simulink model "sm_car_"  (R2026b)
settings: Solver=ode23t  StopTime=100  MaxStep=0.4  AbsTol=1e-3  EnableMultiTasking=on
PreLoadFcn:
  | % Due to usability issue in Repeating Sequence block
  | warning('off','Simulink:Masking:Invalid');
  | 
  | % Eliminate unnecessary warnings in inactive variants
  | % Warnings generated only if you click through inactive variant
  | warning('off','MATLAB:nonExistentField');
  | warning('off','Simulink:Parameters:BlkParamUndefined');
PostLoadFcn:
  | set_param([bdroot '/Vehicle'],'popup_trailer','Off')
  | warning('off','sm:sli:setup:compile:LocalSolverNotSupported')
  | %sm_car_config_maneuver(bdroot,'WOT Braking');
  | sm_car_config_vehicle(bdroot,'false');
  | sm_car_config_logging(bdroot);
InitFcn:
  | sm_car_config_camera;
  | Vehicle = sm_car_vehcfg_checkConfig(Vehicle);
  | sm_car_check_tire_model(bdroot);
StartFcn:
  | tic;
StopFcn:
  | Elapsed_Sim_Time = toc;
  | % disp(['Elapsed Sim Time = ' num2str(Elapsed_Sim_Time)]);
undefined symbols (not defined in the file or in its folder): acc_theta, accel_ramp_rate, Axle1D, AxleIn, Camera, Control, Driver, Init, Maneuver, Pedal, Scene, ShaftL1, ShaftL2, ShaftR1, ShaftR2, Visual, X, xy_data_car_side, Y, Z
libraries: sm_lib x290, fl_lib x171, nesl_utility x144, simulink x60, simulink_extras x14, sdl_lib x14, SimscapeFluids_lib x7, Damper_Element x4, Tire_1x2x x4, ee_lib x3, Scene_Utilities x3, sharedTrackingLibrary x2
(part 18 of 22)

== system sm_car_/Vehicle/Vehicle/Chassis/Damper/Decoupled/Damper A2 Heave ==
  "Ctrl " : Inport
  Linear : Subsystem  VariantControl=Linear  mask(Linear Damper with Bumpstop){dam_b=Damper.Damping.d.Value, hp_dpr_top=Damper.Damping.sTop.Value, hp_dpr_bot=Damper.Damping.sBottom.Value, bs_lim_upper=Damper.Endstop.xMax.Value, bs_lim_lower=Damper.Endstop.xMin.Value, bs_k_upper=Damper.Endstop.KxMax.Value, bs_k_lower=Damper.Endstop.KxMin.Value, bs_b_upper=Damper.Endstop.dxMax.Value, bs_b_lower=Damper.Endstop.dxMin.Value, bs_region=Damper.Endstop.xTransition.Value}
      mask prompts: dam_b "Damper (N/(m/s))"; hp_dpr_top "HP Damper Top [xyz] (m)"; hp_dpr_bot "HP Damper Bottom [xyz] (m)"; bs_region "Transition Region (m)"
      mask help: Linear damper with bumpstop at top and bottom.
      mask init:
      | dam_x0 = norm(hp_dpr_top - hp_dpr_bot);
      mask TypeOptions dam_b: Damper/D
      mask DialogControl text_bumpstop_upper Prompt: Upper
      mask DialogControl text_bumpstop_lower Prompt: Lower
      mask DialogControl text_bumpstop_limit Prompt: Limit (m)
      mask DialogControl text_bumpstop_k Prompt: Stiffness (N/m)
      mask DialogControl text_bumpstop_b Prompt: Damping  (N/(m/s))
  Nonlinear : Subsystem  VariantControl=Nonlinear  mask(Nonlinear Damper with Bumpstop){velocity_vector=Damper.Damping.vDamper.Value, force_vector=Damper.Damping.fDamper.Value, hp_dpr_top=Damper.Damping.sTop.Value, hp_dpr_bot=Damper.Damping.sBottom.Value, bs_lim_upper=Damper.Endstop.xMax.Value, bs_lim_lower=Damper.Endstop.xMin.Value, bs_k_upper=Damper.Endstop.KxMax.Value, bs_k_lower=Damper.Endstop.KxMin.Value, bs_b_upper=Damper.Endstop.dxMax.Value, bs_b_lower=Damper.Endstop.dxMin.Value, bs_region=Damper.Endstop.xTransition.Value}
      mask prompts: velocity_vector "Velocity vector"; force_vector "Force vector"; hp_dpr_top "HP Damper Top [xyz] (m)"; hp_dpr_bot "HP Damper Bottom [xyz] (m)"; bs_region "Transition Region (m)"
      mask help: Damper with damping coefficient specified as a lookup table in parallel with a bumpstop.
      mask init:
      | dam_x0 = norm(hp_dpr_top - hp_dpr_bot);
      mask TypeOptions velocity_vector: Damper/velocity_vector
      mask TypeOptions force_vector: Damper/force_vector
      mask DialogControl text_bumpstop_upper Prompt: Upper
      mask DialogControl text_bumpstop_lower Prompt: Lower
      mask DialogControl text_bumpstop_limit Prompt: Limit (m)
      mask DialogControl text_bumpstop_k Prompt: Stiffness (N/m)
      mask DialogControl text_bumpstop_b Prompt: Damping  (N/(m/s))
  " R" : PMIOPort  Side=Left
  " C" : PMIOPort  Port=2  Side=Right
  " meas" : Outport  VectorParamsAs1DForOutWhenUnconnected=off

== system sm_car_/Vehicle/Vehicle/Chassis/Damper/Decoupled/Damper A2 Roll ==
  "Ctrl " : Inport
  Linear : Subsystem  VariantControl=Linear  mask(Linear Damper with Bumpstop){dam_b=Damper.Damping.d.Value, hp_dpr_top=Damper.Damping.sTop.Value, hp_dpr_bot=Damper.Damping.sBottom.Value, bs_lim_upper=Damper.Endstop.xMax.Value, bs_lim_lower=Damper.Endstop.xMin.Value, bs_k_upper=Damper.Endstop.KxMax.Value, bs_k_lower=Damper.Endstop.KxMin.Value, bs_b_upper=Damper.Endstop.dxMax.Value, bs_b_lower=Damper.Endstop.dxMin.Value, bs_region=Damper.Endstop.xTransition.Value}
      mask prompts: dam_b "Damper (N/(m/s))"; hp_dpr_top "HP Damper Top [xyz] (m)"; hp_dpr_bot "HP Damper Bottom [xyz] (m)"; bs_region "Transition Region (m)"
      mask help: Linear damper with bumpstop at top and bottom.
      mask init:
      | dam_x0 = norm(hp_dpr_top - hp_dpr_bot);
      mask TypeOptions dam_b: Damper/D
      mask DialogControl text_bumpstop_upper Prompt: Upper
      mask DialogControl text_bumpstop_lower Prompt: Lower
      mask DialogControl text_bumpstop_limit Prompt: Limit (m)
      mask DialogControl text_bumpstop_k Prompt: Stiffness (N/m)
      mask DialogControl text_bumpstop_b Prompt: Damping  (N/(m/s))
  Nonlinear : Subsystem  VariantControl=Nonlinear  mask(Nonlinear Damper with Bumpstop){velocity_vector=Damper.Damping.vDamper.Value, force_vector=Damper.Damping.fDamper.Value, hp_dpr_top=Damper.Damping.sTop.Value, hp_dpr_bot=Damper.Damping.sBottom.Value, bs_lim_upper=Damper.Endstop.xMax.Value, bs_lim_lower=Damper.Endstop.xMin.Value, bs_k_upper=Damper.Endstop.KxMax.Value, bs_k_lower=Damper.Endstop.KxMin.Value, bs_b_upper=Damper.Endstop.dxMax.Value, bs_b_lower=Damper.Endstop.dxMin.Value, bs_region=Damper.Endstop.xTransition.Value}
      mask prompts: velocity_vector "Velocity vector"; force_vector "Force vector"; hp_dpr_top "HP Damper Top [xyz] (m)"; hp_dpr_bot "HP Damper Bottom [xyz] (m)"; bs_region "Transition Region (m)"
      mask help: Damper with damping coefficient specified as a lookup table in parallel with a bumpstop.
      mask init:
      | dam_x0 = norm(hp_dpr_top - hp_dpr_bot);
      mask TypeOptions velocity_vector: Damper/velocity_vector
      mask TypeOptions force_vector: Damper/force_vector
      mask DialogControl text_bumpstop_upper Prompt: Upper
      mask DialogControl text_bumpstop_lower Prompt: Lower
      mask DialogControl text_bumpstop_limit Prompt: Limit (m)
      mask DialogControl text_bumpstop_k Prompt: Stiffness (N/m)
      mask DialogControl text_bumpstop_b Prompt: Damping  (N/(m/s))
  " R" : PMIOPort  Side=Left
  " C" : PMIOPort  Port=2  Side=Right
  " meas" : Outport  VectorParamsAs1DForOutWhenUnconnected=off

== system sm_car_/Vehicle/Vehicle/Chassis/Spring/Decoupled/Spring A1 Heave ==
  "Ctrl " : Inport
  Linear : Subsystem  VariantControl=Linear  mask(Linear Spring){spr_def0=Spring.xPreload.Value, spr_k=Spring.K.Value, spr_hp_top=Spring.sTop.Value, spr_hp_bot=Spring.sBottom.Value}
      mask prompts: spr_def0 "Spring Preload (m)"; spr_k "Spring Rate (N/m)"; spr_hp_top "HP Top [xyz] (m)"; spr_hp_bot "HP Bottom [xyz] (m)"
      mask help: Spring with linear stiffness.
      mask init:
      | spr_len0 = norm(spr_hp_top-spr_hp_bot);
  No Spring : Subsystem  VariantControl=No_Spring  mask(No Spring){}
      mask help: Sensor only
  Nonlinear : Subsystem  VariantControl=Nonlinear  mask(Nonlinear Spring){spr_def0=Spring.xPreload.Value, deformation_vector=Spring.xSpring.Value, force_vector=Spring.fSpring.Value, spr_hp_top=Spring.sTop.Value, spr_hp_bot=Spring.sBottom.Value}
      mask prompts: spr_def0 "Spring Preload (m)"; deformation_vector "Deformation vector"; force_vector "Force vector"; spr_hp_top "HP Top [xyz] (m)"; spr_hp_bot "HP Bottom [xyz] (m)"
      mask help: Spring with stiffness specified by a lookup table.
      mask init:
      | spr_len0 = norm(spr_hp_top-spr_hp_bot);
      mask TypeOptions deformation_vector: Spring/deformation_vector
      mask TypeOptions force_vector: Spring/force_vector
  " R" : PMIOPort  Side=Left
  " C" : PMIOPort  Port=2  Side=Right
  " meas" : Outport  VectorParamsAs1DForOutWhenUnconnected=off

== system sm_car_/Vehicle/Vehicle/Chassis/Spring/Decoupled/Spring A1 Roll ==
  "Ctrl " : Inport
  Linear : Subsystem  VariantControl=Linear  mask(Linear Spring){spr_def0=Spring.xPreload.Value, spr_k=Spring.K.Value, spr_hp_top=Spring.sTop.Value, spr_hp_bot=Spring.sBottom.Value}
      mask prompts: spr_def0 "Spring Preload (m)"; spr_k "Spring Rate (N/m)"; spr_hp_top "HP Top [xyz] (m)"; spr_hp_bot "HP Bottom [xyz] (m)"
      mask help: Spring with linear stiffness.
      mask init:
      | spr_len0 = norm(spr_hp_top-spr_hp_bot);
  No Spring : Subsystem  VariantControl=No_Spring  mask(No Spring){}
      mask help: Sensor only
  Nonlinear : Subsystem  VariantControl=Nonlinear  mask(Nonlinear Spring){spr_def0=Spring.xPreload.Value, deformation_vector=Spring.xSpring.Value, force_vector=Spring.fSpring.Value, spr_hp_top=Spring.sTop.Value, spr_hp_bot=Spring.sBottom.Value}
      mask prompts: spr_def0 "Spring Preload (m)"; deformation_vector "Deformation vector"; force_vector "Force vector"; spr_hp_top "HP Top [xyz] (m)"; spr_hp_bot "HP Bottom [xyz] (m)"
      mask help: Spring with stiffness specified by a lookup table.
      mask init:
      | spr_len0 = norm(spr_hp_top-spr_hp_bot);
      mask TypeOptions deformation_vector: Spring/deformation_vector
      mask TypeOptions force_vector: Spring/force_vector
  " R" : PMIOPort  Side=Left
  " C" : PMIOPort  Port=2  Side=Right
  " meas" : Outport  VectorParamsAs1DForOutWhenUnconnected=off

== system sm_car_/Vehicle/Vehicle/Chassis/Spring/Decoupled/Spring A2 Heave ==
  "Ctrl " : Inport
  Linear : Subsystem  VariantControl=Linear  mask(Linear Spring){spr_def0=Spring.xPreload.Value, spr_k=Spring.K.Value, spr_hp_top=Spring.sTop.Value, spr_hp_bot=Spring.sBottom.Value}
      mask prompts: spr_def0 "Spring Preload (m)"; spr_k "Spring Rate (N/m)"; spr_hp_top "HP Top [xyz] (m)"; spr_hp_bot "HP Bottom [xyz] (m)"
      mask help: Spring with linear stiffness.
      mask init:
      | spr_len0 = norm(spr_hp_top-spr_hp_bot);
  No Spring : Subsystem  VariantControl=No_Spring  mask(No Spring){}
      mask help: Sensor only
  Nonlinear : Subsystem  VariantControl=Nonlinear  mask(Nonlinear Spring){spr_def0=Spring.xPreload.Value, deformation_vector=Spring.xSpring.Value, force_vector=Spring.fSpring.Value, spr_hp_top=Spring.sTop.Value, spr_hp_bot=Spring.sBottom.Value}
      mask prompts: spr_def0 "Spring Preload (m)"; deformation_vector "Deformation vector"; force_vector "Force vector"; spr_hp_top "HP Top [xyz] (m)"; spr_hp_bot "HP Bottom [xyz] (m)"
      mask help: Spring with stiffness specified by a lookup table.
      mask init:
      | spr_len0 = norm(spr_hp_top-spr_hp_bot);
      mask TypeOptions deformation_vector: Spring/deformation_vector
      mask TypeOptions force_vector: Spring/force_vector
  " R" : PMIOPort  Side=Left
  " C" : PMIOPort  Port=2  Side=Right
  " meas" : Outport  VectorParamsAs1DForOutWhenUnconnected=off

== system sm_car_/Vehicle/Vehicle/Chassis/Spring/Decoupled/Spring A2 Roll ==
  "Ctrl " : Inport
  Linear : Subsystem  VariantControl=Linear  mask(Linear Spring){spr_def0=Spring.xPreload.Value, spr_k=Spring.K.Value, spr_hp_top=Spring.sTop.Value, spr_hp_bot=Spring.sBottom.Value}
      mask prompts: spr_def0 "Spring Preload (m)"; spr_k "Spring Rate (N/m)"; spr_hp_top "HP Top [xyz] (m)"; spr_hp_bot "HP Bottom [xyz] (m)"
      mask help: Spring with linear stiffness.
      mask init:
      | spr_len0 = norm(spr_hp_top-spr_hp_bot);
  No Spring : Subsystem  VariantControl=No_Spring  mask(No Spring){}
      mask help: Sensor only
  Nonlinear : Subsystem  VariantControl=Nonlinear  mask(Nonlinear Spring){spr_def0=Spring.xPreload.Value, deformation_vector=Spring.xSpring.Value, force_vector=Spring.fSpring.Value, spr_hp_top=Spring.sTop.Value, spr_hp_bot=Spring.sBottom.Value}
      mask prompts: spr_def0 "Spring Preload (m)"; deformation_vector "Deformation vector"; force_vector "Force vector"; spr_hp_top "HP Top [xyz] (m)"; spr_hp_bot "HP Bottom [xyz] (m)"
      mask help: Spring with stiffness specified by a lookup table.
      mask init:
      | spr_len0 = norm(spr_hp_top-spr_hp_bot);
      mask TypeOptions deformation_vector: Spring/deformation_vector
      mask TypeOptions force_vector: Spring/force_vector
  " R" : PMIOPort  Side=Left
  " C" : PMIOPort  Port=2  Side=Right
  " meas" : Outport  VectorParamsAs1DForOutWhenUnconnected=off

== system sm_car_/Vehicle/Vehicle/Chassis/Spring/Independent/Spring L1 ==
  "Ctrl " : Inport
  Linear : Subsystem  VariantControl=Linear  mask(Linear Spring){spr_def0=Spring.xPreload.Value, spr_k=Spring.K.Value, spr_hp_top=Spring.sTop.Value, spr_hp_bot=Spring.sBottom.Value}
      mask prompts: spr_def0 "Spring Preload (m)"; spr_k "Spring Rate (N/m)"; spr_hp_top "HP Top [xyz] (m)"; spr_hp_bot "HP Bottom [xyz] (m)"
      mask help: Spring with linear stiffness.
      mask init:
      | spr_len0 = norm(spr_hp_top-spr_hp_bot);
  " R" : PMIOPort  Side=Left
  " C" : PMIOPort  Port=2  Side=Right
  " meas" : Outport  VectorParamsAs1DForOutWhenUnconnected=off

== system sm_car_/Vehicle/Vehicle/Chassis/Spring/Independent/Spring L2 ==
  "Ctrl " : Inport
  Linear : Subsystem  VariantControl=Linear  mask(Linear Spring){spr_def0=Spring.xPreload.Value, spr_k=Spring.K.Value, spr_hp_top=Spring.sTop.Value, spr_hp_bot=Spring.sBottom.Value}
      mask prompts: spr_def0 "Spring Preload (m)"; spr_k "Spring Rate (N/m)"; spr_hp_top "HP Top [xyz] (m)"; spr_hp_bot "HP Bottom [xyz] (m)"
      mask help: Spring with linear stiffness.
      mask init:
      | spr_len0 = norm(spr_hp_top-spr_hp_bot);
  " R" : PMIOPort  Side=Left
  " C" : PMIOPort  Port=2  Side=Right
  " meas" : Outport  VectorParamsAs1DForOutWhenUnconnected=off

== system sm_car_/Vehicle/Vehicle/Chassis/Spring/Independent/Spring R1 ==
  "Ctrl " : Inport
  Linear : Subsystem  VariantControl=Linear  mask(Linear Spring){spr_def0=Spring.xPreload.Value, spr_k=Spring.K.Value, spr_hp_top=Spring.sTop.Value, spr_hp_bot=Spring.sBottom.Value}
      mask prompts: spr_def0 "Spring Preload (m)"; spr_k "Spring Rate (N/m)"; spr_hp_top "HP Top [xyz] (m)"; spr_hp_bot "HP Bottom [xyz] (m)"
      mask help: Spring with linear stiffness.
      mask init:
      | spr_len0 = norm(spr_hp_top-spr_hp_bot);
  " R" : PMIOPort  Side=Left
  " C" : PMIOPort  Port=2  Side=Right
  " meas" : Outport  VectorParamsAs1DForOutWhenUnconnected=off

== system sm_car_/Vehicle/Vehicle/Chassis/Spring/Independent/Spring R2 ==
  "Ctrl " : Inport
  Linear : Subsystem  VariantControl=Linear  mask(Linear Spring){spr_def0=Spring.xPreload.Value, spr_k=Spring.K.Value, spr_hp_top=Spring.sTop.Value, spr_hp_bot=Spring.sBottom.Value}
      mask prompts: spr_def0 "Spring Preload (m)"; spr_k "Spring Rate (N/m)"; spr_hp_top "HP Top [xyz] (m)"; spr_hp_bot "HP Bottom [xyz] (m)"
      mask help: Spring with linear stiffness.
      mask init:
      | spr_len0 = norm(spr_hp_top-spr_hp_bot);
  " R" : PMIOPort  Side=Left
  " C" : PMIOPort  Port=2  Side=Right
  " meas" : Outport  VectorParamsAs1DForOutWhenUnconnected=off

== system sm_car_/Vehicle/Vehicle/Powertrain/Driveline/L2 R2/Sensing Torque L1 ==
  Ideal Torque Sensor : fl_lib/Mechanical/Mechanical Sensors/Ideal Torque Sensor
  PS-Simulink Converter : nesl_utility/PS-Simulink Converter  PhysicalDomain=network_engine_domain  SubClassName=ps_output  LeftPortType=input  RightPortType=output  PseudoPeriodic=off  Frequencies=[]  VectorFormat=1-D array  Unit=N*m  AffineConversion=off
  C : PMIOPort  Side=Right
  R : PMIOPort  Port=2  Side=Left
  M : Outport  VectorParamsAs1DForOutWhenUnconnected=off
  wires:
  PS-Simulink Converter/1 -> M/1
  connections:
  Ideal Torque Sensor/RConn1 -- C/RConn1
  R/RConn1 -- Ideal Torque Sensor/LConn1
  Ideal Torque Sensor/RConn2 -- PS-Simulink Converter/LConn1

== system sm_car_/Vehicle/Vehicle/Powertrain/Driveline/L2 R2/Sensing Torque L2 ==
  Ideal Torque Sensor : fl_lib/Mechanical/Mechanical Sensors/Ideal Torque Sensor
  PS-Simulink Converter : nesl_utility/PS-Simulink Converter  PhysicalDomain=network_engine_domain  SubClassName=ps_output  LeftPortType=input  RightPortType=output  PseudoPeriodic=off  Frequencies=[]  VectorFormat=1-D array  Unit=N*m  AffineConversion=off
  C : PMIOPort  Side=Right
  R : PMIOPort  Port=2  Side=Left
  M : Outport  VectorParamsAs1DForOutWhenUnconnected=off
  wires:
  PS-Simulink Converter/1 -> M/1
  connections:
  Ideal Torque Sensor/RConn2 -- PS-Simulink Converter/LConn1
  R/RConn1 -- Ideal Torque Sensor/LConn1
  Ideal Torque Sensor/RConn1 -- C/RConn1

== system sm_car_/Vehicle/Vehicle/Powertrain/Driveline/L2 R2/Sensing Torque R1 ==
  Ideal Torque Sensor : fl_lib/Mechanical/Mechanical Sensors/Ideal Torque Sensor
  PS-Simulink Converter : nesl_utility/PS-Simulink Converter  PhysicalDomain=network_engine_domain  SubClassName=ps_output  LeftPortType=input  RightPortType=output  PseudoPeriodic=off  Frequencies=[]  VectorFormat=1-D array  Unit=N*m  AffineConversion=off
  C : PMIOPort  Side=Right
  R : PMIOPort  Port=2  Side=Left
  M : Outport  VectorParamsAs1DForOutWhenUnconnected=off
  wires:
  PS-Simulink Converter/1 -> M/1
  connections:
  Ideal Torque Sensor/RConn2 -- PS-Simulink Converter/LConn1
  R/RConn1 -- Ideal Torque Sensor/LConn1
  Ideal Torque Sensor/RConn1 -- C/RConn1

== system sm_car_/Vehicle/Vehicle/Powertrain/Driveline/L2 R2/Sensing Torque R2 ==
  Ideal Torque Sensor : fl_lib/Mechanical/Mechanical Sensors/Ideal Torque Sensor
  PS-Simulink Converter : nesl_utility/PS-Simulink Converter  PhysicalDomain=network_engine_domain  SubClassName=ps_output  LeftPortType=input  RightPortType=output  PseudoPeriodic=off  Frequencies=[]  VectorFormat=1-D array  Unit=N*m  AffineConversion=off
  C : PMIOPort  Side=Right
  R : PMIOPort  Port=2  Side=Left
  M : Outport  VectorParamsAs1DForOutWhenUnconnected=off
  wires:
  PS-Simulink Converter/1 -> M/1
  connections:
  Ideal Torque Sensor/RConn1 -- C/RConn1
  R/RConn1 -- Ideal Torque Sensor/LConn1
  Ideal Torque Sensor/RConn2 -- PS-Simulink Converter/LConn1

== system sm_car_/Vehicle/Vehicle/Powertrain/Driveline/L2 R2/ShaftL1 ==
  Driveshaft Measurements : Subsystem
  Ideal Torque Sensor : fl_lib/Mechanical/Mechanical Sensors/Ideal Torque Sensor
  No Open Connection : sm_lib/Frames and Transforms/Reference Frame
  PS Terminator : fl_lib/Physical Signals/Sinks/PS Terminator
  Simscape Bus B : SimscapeBus  HierarchyStrings=AxleIn;Axle1D
  Simscape Bus Shaft : SimscapeBus  HierarchyStrings=Shaft1D
  Diff : PMIOPort  Side=Right
  B : PMIOPort  Port=2  Side=Left
  meas : Outport  VectorParamsAs1DForOutWhenUnconnected=off
  wires:
  Driveshaft Measurements/1(meas) -> meas/1
  connections:
  Simscape Bus B/LConn2 -- Ideal Torque Sensor/LConn1
  Ideal Torque Sensor/RConn1 -- Simscape Bus Shaft/LConn1
  Diff/RConn1 -- Simscape Bus Shaft/RConn1
  Ideal Torque Sensor/RConn2 -- PS Terminator/LConn1
  B/RConn1 -- Simscape Bus B/RConn1
  No Open Connection/RConn1 -- Simscape Bus B/LConn1

== system sm_car_/Vehicle/Vehicle/Powertrain/Driveline/L2 R2/ShaftL2 ==
  Ideal Rotational Motion Sensor : fl_lib/Mechanical/Mechanical Sensors/Ideal Rotational Motion Sensor  reference=foundation.enum.MeasurementReference.difference  acceleration_port=false  velocity_port=true  position_port=false  wrap_angle=false  offset=0 rad
  Ideal Torque Sensor : fl_lib/Mechanical/Mechanical Sensors/Ideal Torque Sensor
  Mechanical Rotational Reference : fl_lib/Mechanical/Rotational Elements/Mechanical Rotational Reference
  No Open Connection : sm_lib/Frames and Transforms/Reference Frame
  PS-Simulink Converter : nesl_utility/PS-Simulink Converter  PhysicalDomain=network_engine_domain  SubClassName=ps_output  LeftPortType=input  RightPortType=output  PseudoPeriodic=off  Frequencies=[]  VectorFormat=inherit  Unit=inherit  AffineConversion=off
  PS-Simulink Converter1 : nesl_utility/PS-Simulink Converter  PhysicalDomain=network_engine_domain  SubClassName=ps_output  LeftPortType=input  RightPortType=output  PseudoPeriodic=off  Frequencies=[]  VectorFormat=inherit  Unit=inherit  AffineConversion=off
  Simscape Bus B : SimscapeBus  HierarchyStrings=AxleIn;Axle1D
  Simscape Bus Shaft : SimscapeBus  HierarchyStrings=Shaft1D
  Diff : PMIOPort  Side=Right
  B : PMIOPort  Port=2  Side=Left
  Out Bus Element : Outport  PortName=meas  Element=T
  Out Bus Element1 : Outport  PortName=meas  Element=w
  wires:
  PS-Simulink Converter/1 -> Out Bus Element1/1
  PS-Simulink Converter1/1 -> Out Bus Element/1
  connections:
  Simscape Bus B/LConn2 -- Ideal Rotational Motion Sensor/LConn1 -- Ideal Torque Sensor/LConn1
  Ideal Torque Sensor/RConn1 -- Simscape Bus Shaft/LConn1
  Diff/RConn1 -- Simscape Bus Shaft/RConn1
  Ideal Torque Sensor/RConn2 -- PS-Simulink Converter1/LConn1
  B/RConn1 -- Simscape Bus B/RConn1
  No Open Connection/RConn1 -- Simscape Bus B/LConn1
  Ideal Rotational Motion Sensor/RConn1 -- Mechanical Rotational Reference/LConn1
  Ideal Rotational Motion Sensor/RConn2 -- PS-Simulink Converter/LConn1

== system sm_car_/Vehicle/Vehicle/Powertrain/Driveline/L2 R2/ShaftR1 ==
  Driveshaft Measurements : Subsystem
  Ideal Torque Sensor : fl_lib/Mechanical/Mechanical Sensors/Ideal Torque Sensor
  No Open Connection : sm_lib/Frames and Transforms/Reference Frame
  PS Terminator : fl_lib/Physical Signals/Sinks/PS Terminator
  Simscape Bus B : SimscapeBus  HierarchyStrings=AxleIn;Axle1D
  Simscape Bus Shaft : SimscapeBus  HierarchyStrings=Shaft1D
  Diff : PMIOPort  Side=Right
  B : PMIOPort  Port=2  Side=Left
  meas : Outport  VectorParamsAs1DForOutWhenUnconnected=off
  wires:
  Driveshaft Measurements/1(meas) -> meas/1
  connections:
  Simscape Bus B/LConn2 -- Ideal Torque Sensor/LConn1
  Ideal Torque Sensor/RConn1 -- Simscape Bus Shaft/LConn1
  Diff/RConn1 -- Simscape Bus Shaft/RConn1
  Ideal Torque Sensor/RConn2 -- PS Terminator/LConn1
  B/RConn1 -- Simscape Bus B/RConn1
  No Open Connection/RConn1 -- Simscape Bus B/LConn1

== system sm_car_/Vehicle/Vehicle/Powertrain/Driveline/L2 R2/ShaftR2 ==
  Ideal Rotational Motion Sensor : fl_lib/Mechanical/Mechanical Sensors/Ideal Rotational Motion Sensor  reference=foundation.enum.MeasurementReference.difference  acceleration_port=false  velocity_port=true  position_port=false  wrap_angle=false  offset=0 rad
  Ideal Torque Sensor : fl_lib/Mechanical/Mechanical Sensors/Ideal Torque Sensor
  Mechanical Rotational Reference : fl_lib/Mechanical/Rotational Elements/Mechanical Rotational Reference
  No Open Connection : sm_lib/Frames and Transforms/Reference Frame
  PS-Simulink Converter : nesl_utility/PS-Simulink Converter  PhysicalDomain=network_engine_domain  SubClassName=ps_output  LeftPortType=input  RightPortType=output  PseudoPeriodic=off  Frequencies=[]  VectorFormat=inherit  Unit=inherit  AffineConversion=off
  PS-Simulink Converter1 : nesl_utility/PS-Simulink Converter  PhysicalDomain=network_engine_domain  SubClassName=ps_output  LeftPortType=input  RightPortType=output  PseudoPeriodic=off  Frequencies=[]  VectorFormat=inherit  Unit=inherit  AffineConversion=off
  Simscape Bus B : SimscapeBus  HierarchyStrings=AxleIn;Axle1D
  Simscape Bus Shaft : SimscapeBus  HierarchyStrings=Shaft1D
  Diff : PMIOPort  Side=Right
  B : PMIOPort  Port=2  Side=Left
  Out Bus Element : Outport  PortName=meas  Element=T
  Out Bus Element1 : Outport  PortName=meas  Element=w
  wires:
  PS-Simulink Converter/1 -> Out Bus Element1/1
  PS-Simulink Converter1/1 -> Out Bus Element/1
  connections:
  Simscape Bus B/LConn2 -- Ideal Rotational Motion Sensor/LConn1 -- Ideal Torque Sensor/LConn1
  Ideal Torque Sensor/RConn1 -- Simscape Bus Shaft/LConn1
  Diff/RConn1 -- Simscape Bus Shaft/RConn1
  Ideal Torque Sensor/RConn2 -- PS-Simulink Converter1/LConn1
  B/RConn1 -- Simscape Bus B/RConn1
  No Open Connection/RConn1 -- Simscape Bus B/LConn1
  Ideal Rotational Motion Sensor/RConn2 -- PS-Simulink Converter/LConn1
  Ideal Rotational Motion Sensor/RConn1 -- Mechanical Rotational Reference/LConn1

== system sm_car_/Vehicle/Vehicle/Powertrain/Power/Electric L2 R2/Battery ==
  Battery : batteryecm_lib/Battery (Table-Based)  SOC_vec=Power.Battery.vNoLoad.SOC.Value  T_dependence=simscape.enum.tablebattery.temperature_dependence.yes  prm_dir=simscape.enum.tablebattery.prm_dir.noCurrentDirectionality  T_vec=Power.Battery.vNoLoad.T.Value K  V0_mat=Power.Battery.vNoLoad.V0.Value V  V0_vec=[3.1, 3.27, 3.31, 3.5] V  V_range=[0, inf] V  R0_mat=Power.Battery.rTerminal.R0.Value Ohm  R0_vec=[.015, .017, .012, .013] Ohm  R0_dis_mat=[.03, .015, .002; .04, .017, .008; .039, .012, .006; .027, .013, .021] Ohm  R0_dis_vec=[.015, .017, .012, .013] Ohm  R0_ch_mat=[.03, .015, .002; .04, .017, .008; .039, .012, .006; .027, .013, .021] Ohm  R0_ch_vec=[.015, .017, .012, .013] Ohm  AH=Power.Battery.AhTable.Ah.Value hr*A  prm_leak=1  Rleak_vec=[8000, 7000, 6000] Ohm  Rleak=7e3 Ohm  extrapolation_option=simscape.enum.extrapolation.linear  SOC_port=simscape.enum.tablebattery.enable.yes  prm_dyn=simscape.enum.tablebattery.prm_dyn.off  R1_mat=[.089, .076, .01; .042, .022, .099; .019, .007, .002; .051, .043, .029] Ohm  R1_vec=[.076, .022, .007, .043] Ohm  tau1_mat=[44, 148, 235; 93, 110, 1000; 19, 27, 133; .5, 22, 3] s  tau1_vec=[148, 110, 27, 22] s  R2_mat=[.014, .382, .407; .028, .006, .007; .014, .007, .006; .333, .956, .912] Ohm  R2_vec=[.382, .006, .007, .956] Ohm  tau2_mat=[1, 44, 5644; 11, 24, 506; 2, 14, 330; 3310, 13419, 30216] s  tau2_vec=[44, 24, 14, 13419] s  R3_mat=[.014, .382, .407; .028, .006, .007; .014, .007, .006; .333, .956, .912] Ohm  R3_vec=[.382, .006, .007, .956] Ohm  tau3_mat=[1, 44, 5644; 11, 24, 506; 2, 14, 330; 3310, 13419, 30216] s  tau3_vec=[44, 24, 14, 13419] s  R4_mat=[.014, .382, .407; .028, .006, .007; .014, .007, .006; .333, .956, .912] Ohm  R4_vec=[.382, .006, .007, .956] Ohm  tau4_mat=[1, 44, 5644; 11, 24, 506; 2, 14, 330; 3310, 13419, 30216] s  tau4_vec=[44, 24, 14, 13419] s  R5_mat=[.014, .382, .407; .028, .006, .007; .014, .007, .006; .333, .956, .912] Ohm  R5_vec=[.382, .006, .007, .956] Ohm  tau5_mat=[1, 44, 5644; 11, 24, 506; 2, 14, 330; 3310, 13419, 30216] s  tau5_vec=[44, 24, 14, 13419] s  prm_fade=simscape.enum.tablebattery.prm_fade.equations  N0=100  dV0=0  dR0=0  dAH=0  dRleak=0  dR1=0  dR2=0  dR3=0  dR4=0  dR5=0  N0vec=[100, 200, 300]  Tfadevec=[298.15, 323.15] K  dV0vec=[0, 0, 0]  dR0vec=[0, 0, 0]  dAHvec=[0, 0, 0]  dRleakvec=[0, 0, 0]  dR1vec=[0, 0, 0]  dR2vec=[0, 0, 0]  dR3vec=[0, 0, 0]  dR4vec=[0, 0, 0]  dR5vec=[0, 0, 0]  dV0mat=[0, 0; 0, 0; 0, 0]  dR0mat=[0, 0; 0, 0; 0, 0]  dAHmat=[0, 0; 0, 0; 0, 0]  dRleakmat=[0, 0; 0, 0; 0, 0]  dR1mat=[0, 0; 0, 0; 0, 0]  dR2mat=[0, 0; 0, 0; 0, 0]  dR3mat=[0, 0; 0, 0; 0, 0]  dR4mat=[0, 0; 0, 0; 0, 0]  dR5mat=[0, 0; 0, 0; 0, 0]  prm_age_modeling=simscape.enum.tablebattery.prm_age_modeling.equation  storage_dt_age_vec=[0] d  storage_T_age_vec=[273] K  prm_age_OCV=simscape.enum.tablebattery.prm_age_OCV.OCV  OCV_age=0.9  SOC_age=0.6  prm_age_resistance=simscape.enum.tablebattery.prm_age.disabled  OCV_scaling_age_resistance=2.2134e6  OCV_offset_age_resistance=1.632e6  temp_exp_age_resistance=0.515833569 V  t_exp_age_resistance=0.75  T_age_vec_resistance=[273.15, 298.15, 323.15] K  dt_age_vec_resistance=[90, 180, 270, 360] d  dR0_age_vec=[0, 0, 0]  t_meas_dR0_age=100 d  dR0_age_mat=[0, 0, 0; 0, 0, 0; 0, 0, 0; 0, 0, 0]  prm_age_capacity=simscape.enum.tablebattery.prm_age.disabled  OCV_scaling_age_capacity=1.5097e07  OCV_offset_age_capacity=8.3625e06  temp_exp_age_capacity=0.6011 V  t_exp_age_capacity=0.75  T_age_vec_capacity=[273.15, 298.15, 323.15] K  dt_age_vec_capacity=[90, 180, 270, 360] d  dAH_age_vec=[0, 0, 0]  t_meas_dAH_age=100 d  dAH_age_mat=[0, 0, 0; 0, 0, 0; 0, 0, 0; 0, 0, 0]  thermal_port=simscape.enum.thermaleffects.model  temperature=300 K  thermal_mass=30000 J/K  i_specify=off  i_priority=None  i=0 A  i_nominal_specify=off  i_nominal_value=1  i_nominal_unit=A  v_specify=off  v_priority=None  v=0 V  v_nominal_specify=off  v_nominal_value=1  v_nominal_unit=V  stateOfCharge_specify=on  stateOfCharge_priority=High  stateOfCharge=Power.Battery.SOCInit.Value  stateOfCharge_nominal_specify=off  stateOfCharge_nominal_value=1  stateOfCharge_nominal_unit=1  num_cycles_specify=off  num_cycles_priority=High  num_cycles=0  num_cycles_nominal_specify=off  num_cycles_nominal_value=1  num_cycles_nominal_unit=1  cell_temperature_specify=on  cell_temperature_priority=High  cell_temperature=300 K  cell_temperature_nominal_specify=off  cell_temperature_nominal_value=1  cell_temperature_nominal_unit=K
  Bus Selector : BusSelector  OutputSignals=i,v
  DC-DC Converter : ee_lib/Semiconductors & Converters/Converters/DC-DC Converter  Vref_option=ee.enum.converters.voltageref.internal  v_ref=Power.Converter.vRef.Value V  P_rated=Power.Converter.Power.Value W  droop_enabled=true  droop_param=1  droop=0.001*0 V/A  droop_percent=2  Vref_droop=10 V  reversible=1  G_diode=1e-8 1/Ohm  P_fixed=1 W  losses_option=ee.enum.converters.lossesOption.proportionalToSquaredCurrent  eff_rated=Power.Converter.efficiency.Value  tableOption=ee.enum.converters.lossTableOptionThermal.currentTemp  i_eff_vec=[1, 2, 3, 4] A  v_eff_vec=[15, 30, 45] V  eff_vec=[66, 76, 80, 74]  eff_2D_table=[90, 85, 80; 80, 75, 70; 70, 65, 60; 60, 55, 50]  model_dynamics=1  tau=Power.Converter.fConverter.Value s  v_ini=Power.Converter.vRef.Value V  v1_min=1 V  R1=1000 Ohm  R2=1000 Ohm  T_eff_vec=[280, 300, 320] K  eff_3D_table=repmat([66; 76; 80; 74], 1, 3, 3)  thermal_mass=500 J/K  initial_temperature=25 degC
  ERef Battery : fl_lib/Electrical/Electrical Elements/Electrical Reference
  Filter : simulink_extras/Additional Linear/Transfer Fcn (with initial outputs)  N=[1]  D=[.01 1]  Y0=Power.Battery.SOCInit.Value  U0=0
  Gain2 : Gain  Gain=100
  PS-Simulink Converter3 : nesl_utility/PS-Simulink Converter  PhysicalDomain=network_engine_domain  SubClassName=ps_output  LeftPortType=input  RightPortType=output  PseudoPeriodic=off  Frequencies=[]  VectorFormat=1-D array  Unit=1  AffineConversion=off
  Product1 : Product
  Sensor VI : Subsystem
  To File : ToFile  Commented=on  Filename=SOC_Dej.mat  MatrixName=SOC  SaveFormat=Timeseries
  + : PMIOPort  Side=Right
  - : PMIOPort  Port=2  Side=Right
  HConv : PMIOPort  Port=3  Side=Right
  HBatt : PMIOPort  Port=4  Side=Left
  Out Bus Element5 : Outport  PortName=m  Element=Power
  Out Bus Element6 : Outport  PortName=m  Element=i
  Out Bus Element7 : Outport  PortName=m  Element=v
  Out Bus Element1 : Outport  PortName=m  Element=SOC
  wires:
  Filter/1 -> Gain2/1
  Gain2/1 -> To File/1, Out Bus Element1/1
  PS-Simulink Converter3/1 -> Filter/1
  Bus Selector/1 -> Out Bus Element6/1, Product1/1  "<i>"
  Product1/1 -> Out Bus Element5/1
  Bus Selector/2 -> Product1/2, Out Bus Element7/1  "<v>"
  Sensor VI/1(vi) -> Bus Selector/1
  connections:
  Sensor VI/RConn1 -- DC-DC Converter/LConn1
  Sensor VI/LConn1 -- Battery/LConn1
  HBatt/RConn1 -- Battery/RConn2
  Battery/LConn2 -- PS-Simulink Converter3/LConn1
  +/RConn1 -- DC-DC Converter/RConn1
  Sensor VI/RConn2 -- Battery/RConn1 -- ERef Battery/LConn1 -- DC-DC Converter/LConn2
  -/RConn1 -- DC-DC Converter/RConn2
  HConv/RConn1 -- DC-DC Converter/RConn3

== system sm_car_/Vehicle/Vehicle/Powertrain/Power/Electric L2 R2/Motor L2 ==
  Tr : Inport
  Mechanical Rotational Reference : fl_lib/Mechanical/Rotational Elements/Mechanical Rotational Reference
  Motor : ee_lib/Electromechanical/Motor & Drive (System Level)  torque_speed_param=ee.enum.electromech.envelope.tabulated  overtorque_param=ee.enum.electromech.overtorque.no  T_t=Motor.TorqueSpd.trq.Value N*m  T_t_intermittent=[.36, .32, .28, 0] N*m  T_t_2D=[.09, .09, .09; .08, .08, .08; .07, .07, .07; 0, 0, 0] N*m  T_t_intermittent_2D=[.36, .36, .36; .32, .32, .32; .28, .28, .28; 0, 0, 0] N*m  w_t=Motor.TorqueSpd.w.Value rpm  vdc_t=[6, 12, 24] V  torque_max=0.1 N*m  power_max=30 W  torque_max_intermittent=0.4 N*m  power_max_intermittent=120 W  time_overtorque=30 s  time_recover=60 s  Tc=1/Motor.fActuatorCutoff.Value s  EnableSwitch=false  losses_param=3  eff=100  w_eff=3750 rpm  T_eff=0.08 N*m  Piron=0 W  Pbase=0 W  w_eff_vec=Motor.LossTable.w.Value rpm  T_eff_vec=Motor.LossTable.trq.Value N*m  v_eff_vec=[100, 250, 400] V  losses_mat=[1.49, 1.67, 2.21, 3.1; .42, .69, 1.14, 2.03; .06, .24, .78, 1.68; .42, .69, 1.14, 2.03; 1.49, 1.67, 2.21, 3.1] W  efficiency_mat=Motor.LossTable.efficiency.Value  losses_mat_3D=ones(5, 4, 3) W  efficiency_mat_3D=95 * ones(5, 4, 3)  Res=0 Ohm  J=Motor.J.Value kg*m^2  lam=0 N*m/(rad/s)  speed0=0 rpm  faulted_specify=off  faulted_priority=None  faulted=0  faulted_nominal_specify=off  faulted_nominal_value=1  faulted_nominal_unit=1  isSwitchedOff_specify=off  isSwitchedOff_priority=None  isSwitchedOff=0  isSwitchedOff_nominal_specify=off  isSwitchedOff_nominal_value=1  isSwitchedOff_nominal_unit=1  torqueLimitContinuous_specify=off  torqueLimitContinuous_priority=None  torqueLimitContinuous=0 N*m  torqueLimitContinuous_nominal_specify=off  torqueLimitContinuous_nominal_value=1  torqueLimitContinuous_nominal_unit=N*m  TabulateLossesForMultipleTemperatures=false  alpha=3.93e-3 1/K  Tmeas=Motor.ThermalLoss.T1.Value degC  TmeasVec=[25, 75, 125] degC  Tmeas2=Motor.ThermalLoss.T2.Value degC  losses_mat_T2=[1.49, 1.74, 2.49, 3.74; .42, .67, 1.42, 2.67; .06, .31, 1.06, 2.31; .42, .67, 1.42, 2.67; 1.49, 1.74, 2.49, 3.74] W  efficiency_mat_T2=Motor.ThermalLoss.efficiency.Value  losses_mat_3D_T2=ones(5, 4, 3) W  efficiency_mat_3D_T2=95 * ones(5, 4, 3)  lossesMatMultipleTemperatures=ones(5, 4, 3) W  efficiencyMatMultipleTemperatures=95 * ones(5, 4, 3)  lossesMat4DMultipleTemperatures=ones(5, 4, 3, 3) W  efficiencyMat4DMultipleTemperatures=95 * ones(5, 4, 3, 3)  thermal_mass=Motor.ThermalLoss.mThermal.Value J/K  initial_temperature=Motor.ThermalLoss.Tinit.Value K
  PS-Simulink Converter : nesl_utility/PS-Simulink Converter  PhysicalDomain=network_engine_domain  SubClassName=ps_output  LeftPortType=input  RightPortType=output  PseudoPeriodic=off  Frequencies=[]  VectorFormat=1-D array  Unit=1  AffineConversion=off
  Scope : Scope
      settings: ActiveDisplayYMinimum=-4.02596  ActiveDisplayYMaximum=36.23365
  Scope1 : Scope
      settings: ActiveDisplayYMinimum=-7.5  ActiveDisplayYMaximum=67.5  DataLoggingVariableName=ScopeData2
  Sensing Current : Subsystem
      mask Display: disp('i')
  Sensing Torque : Subsystem
      mask Display: disp('t');
  Simulink-PS Converter2 : nesl_utility/Simulink-PS Converter  PhysicalDomain=network_engine_domain  SubClassName=ps_input  LeftPortType=input  RightPortType=output  PseudoPeriodic=off  Frequencies=[]  NoiseDistribution=none  NoiseParameters=[]  Unit=N*m  AffineConversion=off  FilteringAndDerivatives=provide  SimscapeFilterOrder=1  InputFilterTimeConstant=0.001  UdotUserProvided=0
  + : PMIOPort  Side=Left
  - : PMIOPort  Port=2  Side=Left
  R : PMIOPort  Port=3  Side=Right
  H : PMIOPort  Port=4  Side=Left
  Out Bus Element : Outport  VectorParamsAs1DForOutWhenUnconnected=off  PortName=m  Element=w
  Out Bus Element1 : Outport  VectorParamsAs1DForOutWhenUnconnected=off  PortName=m  Element=trq
  Out Bus Element2 : Outport  VectorParamsAs1DForOutWhenUnconnected=off  PortName=m  Element=i
  wires:
  Sensing Torque/1(T) -> Out Bus Element1/1
  Sensing Current/1(Out1) -> Scope/1, Out Bus Element2/1
  Tr/1 -> Scope1/1, Simulink-PS Converter2/1
  PS-Simulink Converter/1 -> Out Bus Element/1
  connections:
  Sensing Current/LConn1 -- Motor/LConn1
  +/RConn1 -- Sensing Current/RConn1
  Sensing Torque/RConn1 -- R/RConn1
  Sensing Torque/LConn1 -- Motor/LConn3
  Motor/RConn1 -- -/RConn1
  Simulink-PS Converter2/RConn1 -- Motor/LConn2
  Motor/RConn3 -- H/RConn1
  Mechanical Rotational Reference/LConn1 -- Motor/RConn4
  Motor/RConn2 -- PS-Simulink Converter/LConn1

== system sm_car_/Vehicle/Vehicle/Powertrain/Power/Electric L2 R2/Motor R2 ==
  Tr : Inport
  Mechanical Rotational Reference : fl_lib/Mechanical/Rotational Elements/Mechanical Rotational Reference
  Motor : ee_lib/Electromechanical/Motor & Drive (System Level)  torque_speed_param=1  overtorque_param=ee.enum.electromech.overtorque.no  T_t=Motor.TorqueSpd.trq.Value N*m  T_t_intermittent=[.36, .32, .28, 0] N*m  T_t_2D=[.09, .09, .09; .08, .08, .08; .07, .07, .07; 0, 0, 0] N*m  T_t_intermittent_2D=[.36, .36, .36; .32, .32, .32; .28, .28, .28; 0, 0, 0] N*m  w_t=Motor.TorqueSpd.w.Value rpm  vdc_t=[6, 12, 24] V  torque_max=0.1 N*m  power_max=30 W  torque_max_intermittent=0.4 N*m  power_max_intermittent=120 W  time_overtorque=30 s  time_recover=60 s  Tc=1/Motor.fActuatorCutoff.Value s  EnableSwitch=simscape.enum.onoff.off  losses_param=3  eff=100  w_eff=3750 rpm  T_eff=0.08 N*m  Piron=0 W  Pbase=0 W  w_eff_vec=Motor.LossTable.w.Value rpm  T_eff_vec=Motor.LossTable.trq.Value N*m  v_eff_vec=[100, 250, 400] V  losses_mat=[1.49, 1.67, 2.21, 3.1; .42, .69, 1.14, 2.03; .06, .24, .78, 1.68; .42, .69, 1.14, 2.03; 1.49, 1.67, 2.21, 3.1] W  efficiency_mat=Motor.LossTable.efficiency.Value  losses_mat_3D=ones(5, 4, 3) W  efficiency_mat_3D=95 * ones(5, 4, 3)  Res=0 Ohm  J=Motor.J.Value kg*m^2  lam=0 N*m/(rad/s)  speed0=0 rpm  faulted_specify=off  faulted_priority=None  faulted=0  faulted_nominal_specify=off  faulted_nominal_value=1  faulted_nominal_unit=1  isSwitchedOff_specify=off  isSwitchedOff_priority=None  isSwitchedOff=0  isSwitchedOff_nominal_specify=off  isSwitchedOff_nominal_value=1  isSwitchedOff_nominal_unit=1  torqueLimitContinuous_specify=off  torqueLimitContinuous_priority=None  torqueLimitContinuous=0 N*m  torqueLimitContinuous_nominal_specify=off  torqueLimitContinuous_nominal_value=1  torqueLimitContinuous_nominal_unit=N*m  TabulateLossesForMultipleTemperatures=false  alpha=3.93e-3 1/K  Tmeas=Motor.ThermalLoss.T1.Value degC  TmeasVec=[25, 75, 125] degC  Tmeas2=Motor.ThermalLoss.T2.Value degC  losses_mat_T2=[1.49, 1.74, 2.49, 3.74; .42, .67, 1.42, 2.67; .06, .31, 1.06, 2.31; .42, .67, 1.42, 2.67; 1.49, 1.74, 2.49, 3.74] W  efficiency_mat_T2=Motor.ThermalLoss.efficiency.Value  losses_mat_3D_T2=ones(5, 4, 3) W  efficiency_mat_3D_T2=95 * ones(5, 4, 3)  lossesMatMultipleTemperatures=ones(5, 4, 3) W  efficiencyMatMultipleTemperatures=95 * ones(5, 4, 3)  lossesMat4DMultipleTemperatures=ones(5, 4, 3, 3) W  efficiencyMat4DMultipleTemperatures=95 * ones(5, 4, 3, 3)  thermal_mass=Motor.ThermalLoss.mThermal.Value J/K  initial_temperature=Motor.ThermalLoss.Tinit.Value K
  PS-Simulink Converter : nesl_utility/PS-Simulink Converter  PhysicalDomain=network_engine_domain  SubClassName=ps_output  LeftPortType=input  RightPortType=output  PseudoPeriodic=off  Frequencies=[]  VectorFormat=1-D array  Unit=1  AffineConversion=off
  Sensing Current : Subsystem
      mask Display: disp('i')
  Sensing Torque : Subsystem
      mask Display: disp('t');
  Simulink-PS Converter2 : nesl_utility/Simulink-PS Converter  PhysicalDomain=network_engine_domain  SubClassName=ps_input  LeftPortType=input  RightPortType=output  PseudoPeriodic=off  Frequencies=[]  NoiseDistribution=none  NoiseParameters=[]  Unit=N*m  AffineConversion=off  FilteringAndDerivatives=provide  SimscapeFilterOrder=1  InputFilterTimeConstant=0.001  UdotUserProvided=0
  + : PMIOPort  Side=Left
  - : PMIOPort  Port=2  Side=Left
  R : PMIOPort  Port=3  Side=Right
  H : PMIOPort  Port=4  Side=Left
  Out Bus Element : Outport  VectorParamsAs1DForOutWhenUnconnected=off  PortName=m  Element=w
  Out Bus Element1 : Outport  VectorParamsAs1DForOutWhenUnconnected=off  PortName=m  Element=trq
  Out Bus Element2 : Outport  VectorParamsAs1DForOutWhenUnconnected=off  PortName=m  Element=i
  wires:
  Sensing Torque/1(T) -> Out Bus Element1/1
  Sensing Current/1(Out1) -> Out Bus Element2/1
  Tr/1 -> Simulink-PS Converter2/1
  PS-Simulink Converter/1 -> Out Bus Element/1
  connections:
  Sensing Current/LConn1 -- Motor/LConn1
  +/RConn1 -- Sensing Current/RConn1
  Sensing Torque/RConn1 -- R/RConn1
  Sensing Torque/LConn1 -- Motor/LConn3
  Motor/RConn1 -- -/RConn1
  Simulink-PS Converter2/RConn1 -- Motor/LConn2
  Motor/RConn3 -- H/RConn1
  Mechanical Rotational Reference/LConn1 -- Motor/RConn4
  Motor/RConn2 -- PS-Simulink Converter/LConn1

== system sm_car_/Vehicle/Vehicle/Powertrain/Power/Electric L2 R2/Thermal ==
  Liquid Loop1 : Subsystem  VariantControl=Liquid_Loop1
      mask Display: image('sm_car_vehicle_power_cooling_active1loop_IMAGE.png');
  Conv : PMIOPort  Side=Left
  L2 : PMIOPort  Port=2  Side=Left
  R2 : PMIOPort  Port=3  Side=Left
  Ba : PMIOPort  Port=4  Side=Right
  Amb : PMIOPort  Port=5  Side=Right
  " m" : Outport  VectorParamsAs1DForOutWhenUnconnected=off

== system sm_car_/Controller/TrqVec 4Motor/Brake Control/ABS/Sensor/missing tooth/Subsystem ==
  u : Inport
  AND : Logic  AllPortsSameDT=off  OutDataTypeStr=boolean
  FixPt Data Type Duplicate : DataTypeDuplicate  DisableCoverage=on  NumInputPorts=3
  Lower Limit : Constant  DisableCoverage=on  Value=int_limit_lower  OutDataTypeStr=Inherit: Inherit via back propagation
  Lower Test : RelationalOperator  DisableCoverage=on  Operator=<=  OutDataTypeStr=boolean  InputSameDT=off
  Upper Limit : Constant  DisableCoverage=on  Value=int_limit_upper  OutDataTypeStr=Inherit: Inherit via back propagation
  Upper Test : RelationalOperator  DisableCoverage=on  Operator=<=  OutDataTypeStr=boolean  InputSameDT=off
  y : Outport  VectorParamsAs1DForOutWhenUnconnected=off
  wires:
  Lower Limit/1 -> FixPt Data Type Duplicate/2, Lower Test/1
  Upper Limit/1 -> FixPt Data Type Duplicate/3, Upper Test/2
  u/1 -> Upper Test/1, Lower Test/2, FixPt Data Type Duplicate/1
  AND/1 -> y/1
  Upper Test/1 -> AND/2
  Lower Test/1 -> AND/1

== system sm_car_/Controller/TrqVec 4Motor/Brake Control/ABS/Valve Control L1/Categorize Surface/Count Apply Pulses ==
  In1 : Inport
  Trigger : TriggerPort  VariantControl=Variant
  Constant : Constant  Value=0
  Memory : Memory  InheritSampleTime=on
  Pulse Increment : Constant
  Sum : Sum  Inputs=|++
  Switch : Switch  Criteria=u2 > Threshold  Threshold=0.5  ZeroCross=off  SaturateOnIntegerOverflow=off  InputSameDT=off
  Apply Pulses : Outport  VectorParamsAs1DForOutWhenUnconnected=off
  wires:
  Pulse Increment/1 -> Sum/2
  Sum/1 -> Switch/3, Apply Pulses/1
  Memory/1 -> Sum/1
  In1/1 -> Switch/2
  Constant/1 -> Switch/1
  Switch/1 -> Memory/1

== system sm_car_/Controller/TrqVec 4Motor/Brake Control/ABS/Valve Control L1/Categorize Surface/Total Apply Pulses This Cycle ==
  In1 : Inport
  Trigger : TriggerPort  VariantControl=Variant
  Total Pulses : Outport  VectorParamsAs1DForOutWhenUnconnected=off
  wires:
  In1/1 -> Total Pulses/1

== system sm_car_/Controller/TrqVec 4Motor/Brake Control/ABS/Valve Control L2/Categorize Surface/Count Apply Pulses ==
  In1 : Inport
  Trigger : TriggerPort  VariantControl=Variant
  Constant : Constant  Value=0
  Memory : Memory  InheritSampleTime=on
  Pulse Increment : Constant
  Sum : Sum  Inputs=|++
  Switch : Switch  Criteria=u2 > Threshold  Threshold=0.5  ZeroCross=off  SaturateOnIntegerOverflow=off  InputSameDT=off
  Apply Pulses : Outport  VectorParamsAs1DForOutWhenUnconnected=off
  wires:
  Pulse Increment/1 -> Sum/2
  Sum/1 -> Switch/3, Apply Pulses/1
  Memory/1 -> Sum/1
  In1/1 -> Switch/2
  Constant/1 -> Switch/1
  Switch/1 -> Memory/1

== system sm_car_/Controller/TrqVec 4Motor/Brake Control/ABS/Valve Control L2/Categorize Surface/Total Apply Pulses This Cycle ==
  In1 : Inport
  Trigger : TriggerPort  VariantControl=Variant
  Total Pulses : Outport  VectorParamsAs1DForOutWhenUnconnected=off
  wires:
  In1/1 -> Total Pulses/1

== system sm_car_/Controller/TrqVec 4Motor/Brake Control/ABS/Valve Control R1/Categorize Surface/Count Apply Pulses ==
  In1 : Inport
  Trigger : TriggerPort  VariantControl=Variant
  Constant : Constant  Value=0
  Memory : Memory  InheritSampleTime=on
  Pulse Increment : Constant
  Sum : Sum  Inputs=|++
  Switch : Switch  Criteria=u2 > Threshold  Threshold=0.5  ZeroCross=off  SaturateOnIntegerOverflow=off  InputSameDT=off
  Apply Pulses : Outport  VectorParamsAs1DForOutWhenUnconnected=off
  wires:
  Pulse Increment/1 -> Sum/2
  Sum/1 -> Switch/3, Apply Pulses/1
  Memory/1 -> Sum/1
  In1/1 -> Switch/2
  Constant/1 -> Switch/1
  Switch/1 -> Memory/1

== system sm_car_/Controller/TrqVec 4Motor/Brake Control/ABS/Valve Control R1/Categorize Surface/Total Apply Pulses This Cycle ==
  In1 : Inport
  Trigger : TriggerPort  VariantControl=Variant
  Total Pulses : Outport  VectorParamsAs1DForOutWhenUnconnected=off
  wires:
  In1/1 -> Total Pulses/1

== system sm_car_/Controller/TrqVec 4Motor/Brake Control/ABS/Valve Control R2/Categorize Surface/Count Apply Pulses ==
  In1 : Inport
  Trigger : TriggerPort  VariantControl=Variant
  Constant : Constant  Value=0
  Memory : Memory  InheritSampleTime=on
  Pulse Increment : Constant
  Sum : Sum  Inputs=|++
  Switch : Switch  Criteria=u2 > Threshold  Threshold=0.5  ZeroCross=off  SaturateOnIntegerOverflow=off  InputSameDT=off
  Apply Pulses : Outport  VectorParamsAs1DForOutWhenUnconnected=off
  wires:
  Pulse Increment/1 -> Sum/2
  Sum/1 -> Switch/3, Apply Pulses/1
  Memory/1 -> Sum/1
  In1/1 -> Switch/2
  Constant/1 -> Switch/1
  Switch/1 -> Memory/1

== system sm_car_/Controller/TrqVec 4Motor/Brake Control/ABS/Valve Control R2/Categorize Surface/Total Apply Pulses This Cycle ==
  In1 : Inport
  Trigger : TriggerPort  VariantControl=Variant
  Total Pulses : Outport  VectorParamsAs1DForOutWhenUnconnected=off
  wires:
  In1/1 -> Total Pulses/1
